simulink model "Friction_ramp"  (R2025b)
settings: Solver=FixedStepDiscrete  StartTime=0.0  StopTime=50  FixedStep=1e-4  RelTol=1e-3
undefined symbols (not defined in the file or in its folder): Pull, up
libraries: speedgoatlib_IO183 x3
settings Model: SimulationMode=external  Creator=rafaeltavares  LastModifiedBy=havard
settings SolverCC: ConcurrentTasks=on  AlgebraicLoopSolver=TrustRegion  PositivePriorityOrder=on  InsertRTBMode=Never (minimum delay)
settings DataIOCC: SaveFormat=StructureWithTime  ReturnWorkspaceOutputs=off
settings OptimizationCC: BlockReduction=off  OptimizeBlockIOStorage=off  BufferReuse=off  GlobalBufferReuse=off  ExpressionFolding=off  LocalBlockOutputs=off  OptimizeDataStoreBuffers=off  BusAssignmentInplaceUpdate=off
settings DebuggingCC: TasksWithSamePriorityMsg=none  UnconnectedInputMsg=warning  UnconnectedOutputMsg=warning  UnconnectedLineMsg=warning  UnderSpecifiedDimensionMsg=warning  ArithmeticOperatorsInVariantConditions=warning
settings HardwareCC: ProdBitPerLong=64.0  ProdLongLongMode=on  ProdHWDeviceType=Intel->x86-64 (Linux 64)
settings ModelReferenceCC: EnableRefExpFcnMdlSchedulingChecks=on
settings SFSimCC: CustomCodeUndefinedFunction=UseInterfaceOnly
settings RTWCC: SystemTargetFile=speedgoat.tlc  TemplateMakefile=slrealtime_default_tmf  Toolchain=Simulink Real-Time Toolchain  BuildConfiguration=Faster Runs  CodeExecutionProfiling=on  TargetLang=C++  GPUComputeCapability=3.5  DLArmComputeVersion=19.05  Description=Speedgoat Real-Time Target Machine
settings SimulinkRealTimeTargetCC: SLRTFileLogMaxRuns=1.0  ExtModeMaxTrigDuration=10.0  ExtModeStaticAllocSize=1000000.0  ExtModeTransport=0.0  MultiwordLength=2048.0  DynamicStringBufferSize=256.0  PreserveMATLABNamespacesInGeneratedCode=on  SubcomponentCodeInterfacePackaging=Reusable function  InstructionSetFMA=off  LogToMDFFile=off

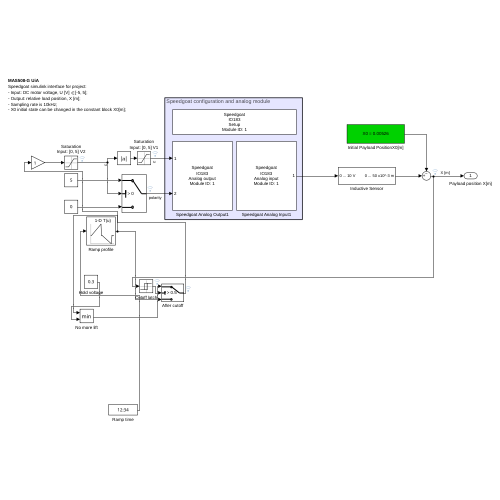
[thumbnail: Simulink's stored preview of the top-level diagram]
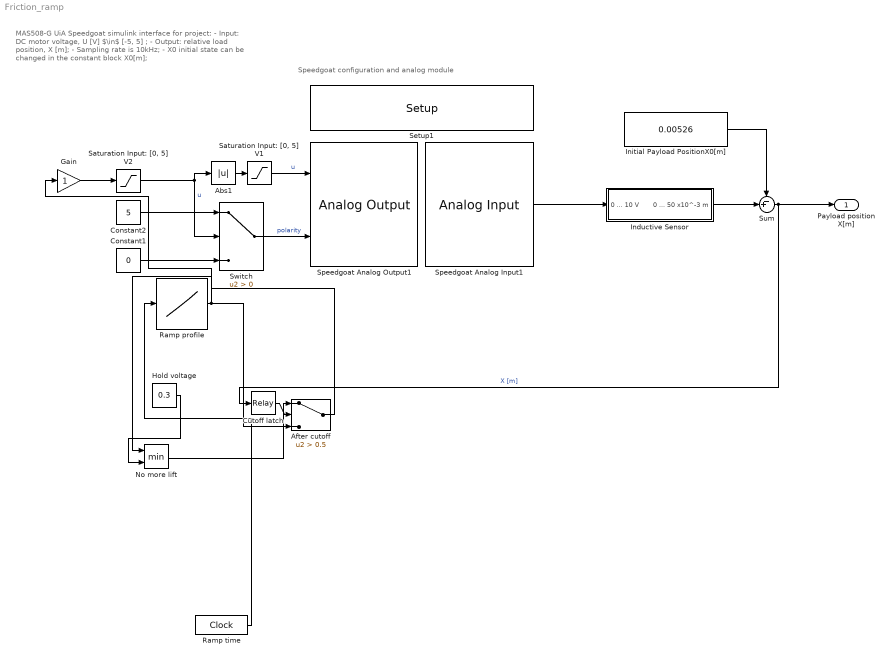
== system Friction_ramp ==
  note: MAS508-G UiA
      | Speedgoat simulink interface for project:
      | - Input: DC motor voltage, U [V] $\in$ [-5, 5] ;
      | - Output: relative load position, X [m];
      | - Sampling rate is 10kHz;
      | - X0 initial state can be changed in the constant block X0[m];
  note: Speedgoat configuration and analog module
  Abs1 : Abs  SaturateOnIntegerOverflow=off
  After cutoff : Switch  Criteria=u2 > Threshold  Threshold=0.5  SaturateOnIntegerOverflow=off  InputSameDT=off
  Constant1 : Constant  Value=0
  Constant2 : Constant  Value=5
  Cutoff latch : Relay  OnSwitchValue=0.012  OffSwitchValue=-1
  Gain : Gain
  Hold voltage : Constant  Value=0.3
  "Inductive Sensor " : Subsystem
  "Initial Payload PositionX0[m] " : Constant  Value=0.00526
      mask Display:
      | set_param(gcb,'BackgroundColor','green');
      | fprintf('X0 = %s', get_param(gcb,'Value'))
  No more lift : MinMax  Inputs=2
  Ramp profile : Lookup_n-D  NumberOfTableDimensions=1  BreakpointsForDimension1=[0 2 22 23 24 44 46 50]  Table=[0.3 0.3 1.5 0.3 0.3 -0.6 0.3 0.3]  ExtrapMethod=Clip  InternalRulePriority=Speed  RndMeth=Simplest
  Ramp time : DigitalClock  SampleTime=1e-4
  "Saturation Input: [0, 5] V1" : Saturate  UpperLimit=5  LowerLimit=0
  "Saturation Input: [0, 5] V2" : Saturate  UpperLimit=5  LowerLimit=-5
  Setup1 : speedgoatlib_IO183/Setup  parModuleId=1  parPciSlot=-1  parDaSimult=on  parAdCoupling=Single Ended  parAdRange=0..10V  parAdChannelLow=1  parAdChannelHigh=1  parDaChannels=[1 2]  parDaRange=0..5V  parDaInit=[0 5 0 0]  parDaReset=1  parDoChannels=[1:8]  parDoInit=[0]  parDoReset=[1]  parDiChannels=[9:16]  parIOPullReferenceFront=Pull-up (3.3V)  parIOPullReferenceRear=Pull-up (3.3V)
      settings: SourceProductName=IO183
  Speedgoat Analog Input1 : speedgoatlib_IO183/Analog Input  Priority=0  parModuleId=1  parSampTime=-1  parPciSlot=-1  parAdChannelLow=1  parAdChannelHigh=1
      settings: SourceProductName=IO183
  Speedgoat Analog Output1 : speedgoatlib_IO183/Analog Output  parModuleId=1  parSampTime=-1  parDaSimult=on  parPciSlot=-1  parDaChannels=[1 2]  parDaInit=[0 5 0 0]  parDaReset=[1 1 1 1]
      settings: SourceProductName=IO183
  Sum : Sum  Inputs=-+|
  Switch : Switch  Criteria=u2 > Threshold  SaturateOnIntegerOverflow=off  InputSameDT=off
  Payload position X[m] : Outport
  wires:
  "Inductive Sensor "/1(0 ... 50 x10^-3 m) -> Sum/2
  "Initial Payload PositionX0[m] "/1 -> Sum/1
  "Saturation Input: [0, 5] V1"/1 -> Speedgoat Analog Output1/1  "u"
  Constant2/1 -> Switch/1
  Speedgoat Analog Input1/1 -> "Inductive Sensor "/1(0 ... 10 V)
  Abs1/1 -> "Saturation Input: [0, 5] V1"/1
  Switch/1 -> Speedgoat Analog Output1/2  "polarity"
  Constant1/1 -> Switch/3
  Gain/1 -> "Saturation Input: [0, 5] V2"/1
  "Saturation Input: [0, 5] V2"/1 -> Switch/2, Abs1/1  "u"
  Sum/1 -> Payload position X[m]/1, Cutoff latch/1  "X [m]"
  Ramp time/1 -> Ramp profile/1
  Ramp profile/1 -> No more lift/1, After cutoff/3
  Hold voltage/1 -> No more lift/2
  No more lift/1 -> After cutoff/1
  Cutoff latch/1 -> After cutoff/2
  After cutoff/1 -> Gain/1

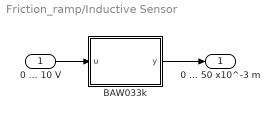
== system Friction_ramp/Inductive Sensor  ==
  0 ... 10 V : Inport
  BAW033k : MATLAB Function  TreatAsAtomicUnit=on
  0 ... 50 x10^-3 m : Outport  VectorParamsAs1DForOutWhenUnconnected=off
  wires:
  BAW033k/1(y) -> 0 ... 50 x10^-3 m/1
  0 ... 10 V/1 -> BAW033k/1(u)

== matlab function Friction_ramp/Inductive Sensor /BAW033k ==
  data: u input; y output
function y = fcn(u)
% Input: 0 ... 10 V
% Output: 0 ... 40 mm
y =(40*10^-3/10)*u; %Output in SI [m]
